simulink model "ASM_Traffic_A11"  (R2026a)
settings: Solver=ode1  StartTime=SIM.tstart.v  StopTime=SIM.tend.v  FixedStep=SIM.StepSize.v
PostLoadFcn:
  | if any(exist('dsrtsu_mdlpostloadfcn', 'file') ~= 0), dsrtsu_mdlpostloadfcn('Execute', bdroot); end
  | try, asm_mdl_postloadfcn(bdroot, 'UpdateModel', 3600); catch, disp(lasterr); end,
InitFcn:
  | , if any(exist('rtifpga_mdlclblib', 'file') ~= 0), rtifpga_mdlclblib('Init', bdroot); end,
  | , if any(exist('dsmpb_private', 'file') ~= 0), dsmpb_private('dsmpb_mdlclblib', 'Init', bdroot); end,
undefined symbols (not defined in the file): _to_, a0b2, ASM_BrakeHydraulics_DemoSystems, ASM_VehicleDynamics_DemoSystems, b98103fe8ad365046cd0, BrakeCircuit, controllerConfig, CPT, Crankshaft, DiscIntNeverNeededParam, dsmsi, FinalDriveAssembly, instance, MDL, ModeSignals, mu, Pos_BrakePedal_Maneuver, rad, RefSignals, s_to_rpm, SIM, SoftECU, Suspension, Tire, Transmission
libraries: ASM_Traffic_lib x135, simulink x98, ASM_Utils_lib x77, ASM_VehicleDynamics_lib x70, ASM_Environment_lib x22, dsmpblib x20, dsmsilib x15, MDLD_Utils_lib x10, ASM_BrakeHydraulics_lib x3, sl_discontinuities x2
(part 19 of 63)

== system ASM_Traffic_A11/Driver/Interface_In/ModelSignals/Mode_AcceleratorBrake[1Stim|2Driver]_ ==
  In1 : Inport
  DummyGain : Gain  SaturateOnIntegerOverflow=on  OutDataTypeStr=Inherit: Same as input  ParamDataTypeStr=Inherit: Same as input
  Out1 : Outport  VectorParamsAs1DForOutWhenUnconnected=off
  wires:
  In1/1 -> DummyGain/1
  DummyGain/1 -> Out1/1

== system ASM_Traffic_A11/Driver/Interface_In/ModelSignals/Mode_AdaptVelocityToRoad[1Off|2On]_ ==
  In1 : Inport
  Gain : Gain  SaturateOnIntegerOverflow=on  OutDataTypeStr=Inherit: Same as input  ParamDataTypeStr=Inherit: Same as input
  Out1 : Outport  VectorParamsAs1DForOutWhenUnconnected=off
  wires:
  In1/1 -> Gain/1
  Gain/1 -> Out1/1

== system ASM_Traffic_A11/Driver/Interface_In/ModelSignals/Mode_CurvatureCalculation[1Road|2Driver]_ ==
  In1 : Inport
  Gain : Gain  SaturateOnIntegerOverflow=on  OutDataTypeStr=Inherit: Same as input  ParamDataTypeStr=Inherit: Same as input
  Out1 : Outport  VectorParamsAs1DForOutWhenUnconnected=off
  wires:
  In1/1 -> Gain/1
  Gain/1 -> Out1/1

== system ASM_Traffic_A11/Driver/Interface_In/ModelSignals/Mode_ForceToRoad[1Off|2On]_ ==
  In1 : Inport
  Gain : Gain  SaturateOnIntegerOverflow=on  OutDataTypeStr=Inherit: Same as input  ParamDataTypeStr=Inherit: Same as input
  Out1 : Outport  VectorParamsAs1DForOutWhenUnconnected=off
  wires:
  Gain/1 -> Out1/1
  In1/1 -> Gain/1

== system ASM_Traffic_A11/Driver/Interface_In/ModelSignals/Mode_GearClutch[1Stim|2Driver|3OpenClutch|4RefGear]_ ==
  In1 : Inport
  DummyGain : Gain  SaturateOnIntegerOverflow=on  OutDataTypeStr=Inherit: Same as input  ParamDataTypeStr=Inherit: Same as input
  Out1 : Outport  VectorParamsAs1DForOutWhenUnconnected=off
  wires:
  In1/1 -> DummyGain/1
  DummyGain/1 -> Out1/1

== system ASM_Traffic_A11/Driver/Interface_In/ModelSignals/Mode_LatCtrl[1Pos|2Yaw]_ ==
  In1 : Inport
  Gain : Gain  SaturateOnIntegerOverflow=on  OutDataTypeStr=Inherit: Same as input  ParamDataTypeStr=Inherit: Same as input
  Out1 : Outport  VectorParamsAs1DForOutWhenUnconnected=off
  wires:
  Gain/1 -> Out1/1
  In1/1 -> Gain/1

== system ASM_Traffic_A11/Driver/Interface_In/ModelSignals/Mode_SelectorLever[1Stim|2Driver]_ ==
  In1 : Inport
  Gain : Gain  SaturateOnIntegerOverflow=on  OutDataTypeStr=Inherit: Same as input  ParamDataTypeStr=Inherit: Same as input
  Out1 : Outport  VectorParamsAs1DForOutWhenUnconnected=off
  wires:
  In1/1 -> Gain/1
  Gain/1 -> Out1/1

== system ASM_Traffic_A11/Driver/Interface_In/ModelSignals/Mode_Steer[1Stim|2Driver|3Fix]_ ==
  In1 : Inport
  Gain : Gain  SaturateOnIntegerOverflow=on  OutDataTypeStr=Inherit: Same as input  ParamDataTypeStr=Inherit: Same as input
  Out1 : Outport  VectorParamsAs1DForOutWhenUnconnected=off
  wires:
  In1/1 -> Gain/1
  Gain/1 -> Out1/1

== system ASM_Traffic_A11/Driver/Interface_In/ModelSignals/Mode_TrafficDriver[1Off|2On]_ ==
  In1 : Inport
  Gain : Gain  SaturateOnIntegerOverflow=on  OutDataTypeStr=Inherit: Same as input  ParamDataTypeStr=Inherit: Same as input
  Out1 : Outport  VectorParamsAs1DForOutWhenUnconnected=off
  wires:
  Gain/1 -> Out1/1
  In1/1 -> Gain/1

== system ASM_Traffic_A11/Driver/Interface_In/ModelSignals/Mode_Transmission[1Manual|2Automatic]_ ==
  In1 : Inport
  DummyGain : Gain  SaturateOnIntegerOverflow=on  OutDataTypeStr=Inherit: Same as input  ParamDataTypeStr=Inherit: Same as input
  Out1 : Outport  VectorParamsAs1DForOutWhenUnconnected=off
  wires:
  In1/1 -> DummyGain/1
  DummyGain/1 -> Out1/1

== system ASM_Traffic_A11/Driver/Interface_In/ModelSignals/Pitch_Preview_Road[deg]_ ==
  In1 : Inport
  Gain : Gain  SaturateOnIntegerOverflow=on  OutDataTypeStr=Inherit: Same as input  ParamDataTypeStr=Inherit: Same as input
  Out1 : Outport  VectorParamsAs1DForOutWhenUnconnected=off
  wires:
  Gain/1 -> Out1/1
  In1/1 -> Gain/1

== system ASM_Traffic_A11/Driver/Interface_In/ModelSignals/Pos_AccPedal_Maneuver[%]_ ==
  In1 : Inport
  DummyGain : Gain  SaturateOnIntegerOverflow=on  OutDataTypeStr=Inherit: Same as input  ParamDataTypeStr=Inherit: Same as input
  Out1 : Outport  VectorParamsAs1DForOutWhenUnconnected=off
  wires:
  In1/1 -> DummyGain/1
  DummyGain/1 -> Out1/1

== system ASM_Traffic_A11/Driver/Interface_In/ModelSignals/Pos_BrakePedal_Maneuver[%]_ ==
  In1 : Inport
  DummyGain : Gain  SaturateOnIntegerOverflow=on  OutDataTypeStr=Inherit: Same as input  ParamDataTypeStr=Inherit: Same as input
  Out1 : Outport  VectorParamsAs1DForOutWhenUnconnected=off
  wires:
  In1/1 -> DummyGain/1
  DummyGain/1 -> Out1/1

== system ASM_Traffic_A11/Driver/Interface_In/ModelSignals/Pos_ClutchPedal_Maneuver[%]_ ==
  In1 : Inport
  DummyGain : Gain  SaturateOnIntegerOverflow=on  OutDataTypeStr=Inherit: Same as input  ParamDataTypeStr=Inherit: Same as input
  Out1 : Outport  VectorParamsAs1DForOutWhenUnconnected=off
  wires:
  In1/1 -> DummyGain/1
  DummyGain/1 -> Out1/1

== system ASM_Traffic_A11/Driver/Interface_In/ModelSignals/Pos_x_CoG_Vehicle_Total[m]_ ==
  In1 : Inport
  DummyGain : Gain  SaturateOnIntegerOverflow=on  OutDataTypeStr=Inherit: Same as input  ParamDataTypeStr=Inherit: Same as input
  Out1 : Outport  VectorParamsAs1DForOutWhenUnconnected=off
  wires:
  In1/1 -> DummyGain/1
  DummyGain/1 -> Out1/1

== system ASM_Traffic_A11/Driver/Interface_In/ModelSignals/Pos_x_Preview_DriverCurv[m]_ ==
  In1 : Inport
  Gain : Gain  SaturateOnIntegerOverflow=on  OutDataTypeStr=Inherit: Same as input  ParamDataTypeStr=Inherit: Same as input
  Out1 : Outport  VectorParamsAs1DForOutWhenUnconnected=off
  wires:
  In1/1 -> Gain/1
  Gain/1 -> Out1/1

== system ASM_Traffic_A11/Driver/Interface_In/ModelSignals/Pos_x_Preview_Road[m]_ ==
  In1 : Inport
  Gain : Gain  SaturateOnIntegerOverflow=on  OutDataTypeStr=Inherit: Same as input  ParamDataTypeStr=Inherit: Same as input
  Out1 : Outport  VectorParamsAs1DForOutWhenUnconnected=off
  wires:
  Gain/1 -> Out1/1
  In1/1 -> Gain/1

== system ASM_Traffic_A11/Driver/Interface_In/ModelSignals/Pos_x_Ref_Vehicle_Road[m]_ ==
  In1 : Inport
  Gain : Gain  SaturateOnIntegerOverflow=on  OutDataTypeStr=Inherit: Same as input  ParamDataTypeStr=Inherit: Same as input
  Out1 : Outport  VectorParamsAs1DForOutWhenUnconnected=off
  wires:
  Gain/1 -> Out1/1
  In1/1 -> Gain/1

== system ASM_Traffic_A11/Driver/Interface_In/ModelSignals/Pos_x_Vehicle_CoorSys_E[m]_ ==
  In1 : Inport
  DummyGain : Gain  SaturateOnIntegerOverflow=on  OutDataTypeStr=Inherit: Same as input  ParamDataTypeStr=Inherit: Same as input
  Out1 : Outport  VectorParamsAs1DForOutWhenUnconnected=off
  wires:
  In1/1 -> DummyGain/1
  DummyGain/1 -> Out1/1

== system ASM_Traffic_A11/Driver/Interface_In/ModelSignals/Pos_y_Preview_DriverCurv[m]_ ==
  In1 : Inport
  Gain : Gain  SaturateOnIntegerOverflow=on  OutDataTypeStr=Inherit: Same as input  ParamDataTypeStr=Inherit: Same as input
  Out1 : Outport  VectorParamsAs1DForOutWhenUnconnected=off
  wires:
  Gain/1 -> Out1/1
  In1/1 -> Gain/1

== system ASM_Traffic_A11/Driver/Interface_In/ModelSignals/Pos_y_Preview_Road[m]_ ==
  In1 : Inport
  Gain : Gain  SaturateOnIntegerOverflow=on  OutDataTypeStr=Inherit: Same as input  ParamDataTypeStr=Inherit: Same as input
  Out1 : Outport  VectorParamsAs1DForOutWhenUnconnected=off
  wires:
  In1/1 -> Gain/1
  Gain/1 -> Out1/1

== system ASM_Traffic_A11/Driver/Interface_In/ModelSignals/Pos_y_Ref_Vehicle_Road[m]_ ==
  In1 : Inport
  Gain : Gain  SaturateOnIntegerOverflow=on  OutDataTypeStr=Inherit: Same as input  ParamDataTypeStr=Inherit: Same as input
  Out1 : Outport  VectorParamsAs1DForOutWhenUnconnected=off
  wires:
  In1/1 -> Gain/1
  Gain/1 -> Out1/1

== system ASM_Traffic_A11/Driver/Interface_In/ModelSignals/Pos_y_Vehicle_CoorSys_E[m]_ ==
  In1 : Inport
  DummyGain : Gain  SaturateOnIntegerOverflow=on  OutDataTypeStr=Inherit: Same as input  ParamDataTypeStr=Inherit: Same as input
  Out1 : Outport  VectorParamsAs1DForOutWhenUnconnected=off
  wires:
  DummyGain/1 -> Out1/1
  In1/1 -> DummyGain/1

== system ASM_Traffic_A11/Driver/Interface_In/ModelSignals/Pos_z_Preview_Road[m]_ ==
  In1 : Inport
  Gain : Gain  SaturateOnIntegerOverflow=on  OutDataTypeStr=Inherit: Same as input  ParamDataTypeStr=Inherit: Same as input
  Out1 : Outport  VectorParamsAs1DForOutWhenUnconnected=off
  wires:
  Gain/1 -> Out1/1
  In1/1 -> Gain/1

== system ASM_Traffic_A11/Driver/Interface_In/ModelSignals/Reset_States[0|1]_ ==
  In1 : Inport
  DummyGain : Gain  SaturateOnIntegerOverflow=on  OutDataTypeStr=Inherit: Same as input  ParamDataTypeStr=Inherit: Same as input
  Out1 : Outport  VectorParamsAs1DForOutWhenUnconnected=off
  wires:
  DummyGain/1 -> Out1/1
  In1/1 -> DummyGain/1

== system ASM_Traffic_A11/Driver/Interface_In/ModelSignals/Roll_Preview_Road[deg]_ ==
  In1 : Inport
  Gain : Gain  SaturateOnIntegerOverflow=on  OutDataTypeStr=Inherit: Same as input  ParamDataTypeStr=Inherit: Same as input
  Out1 : Outport  VectorParamsAs1DForOutWhenUnconnected=off
  wires:
  In1/1 -> Gain/1
  Gain/1 -> Out1/1

== system ASM_Traffic_A11/Driver/Interface_In/ModelSignals/Route_Direction_Init[]_ ==
  In1 : Inport
  Gain : Gain  SaturateOnIntegerOverflow=on  OutDataTypeStr=Inherit: Same as input  ParamDataTypeStr=Inherit: Same as input
  Out1 : Outport  VectorParamsAs1DForOutWhenUnconnected=off
  wires:
  Gain/1 -> Out1/1
  In1/1 -> Gain/1

== system ASM_Traffic_A11/Driver/Interface_In/ModelSignals/SelectorLever_Maneuver[-3T|-2P|-1R|0N|1D]_ ==
  In1 : Inport
  DummyGain : Gain  SaturateOnIntegerOverflow=on  OutDataTypeStr=Inherit: Same as input  ParamDataTypeStr=Inherit: Same as input
  Out1 : Outport  VectorParamsAs1DForOutWhenUnconnected=off
  wires:
  In1/1 -> DummyGain/1
  DummyGain/1 -> Out1/1

== system ASM_Traffic_A11/Driver/Interface_In/ModelSignals/Speed_Limit_Preview_Road[km|h]_ ==
  In1 : Inport
  Gain : Gain  SaturateOnIntegerOverflow=on  OutDataTypeStr=Inherit: Same as input  ParamDataTypeStr=Inherit: Same as input
  Out1 : Outport  VectorParamsAs1DForOutWhenUnconnected=off
  wires:
  In1/1 -> Gain/1
  Gain/1 -> Out1/1

== system ASM_Traffic_A11/Driver/Interface_In/ModelSignals/State_Engine[0|1|2|3|4]_ ==
  In1 : Inport
  DummyGain : Gain  SaturateOnIntegerOverflow=on  OutDataTypeStr=Inherit: Same as input  ParamDataTypeStr=Inherit: Same as input
  Out1 : Outport  VectorParamsAs1DForOutWhenUnconnected=off
  wires:
  DummyGain/1 -> Out1/1
  In1/1 -> DummyGain/1

== system ASM_Traffic_A11/Driver/Interface_In/ModelSignals/State_StartStop[1Off|2NotReady|3Ready|4EngStopped]_ ==
  In1 : Inport
  DummyGain : Gain  SaturateOnIntegerOverflow=on  OutDataTypeStr=Inherit: Same as input  ParamDataTypeStr=Inherit: Same as input
  Out1 : Outport  VectorParamsAs1DForOutWhenUnconnected=off
  wires:
  In1/1 -> DummyGain/1
  DummyGain/1 -> Out1/1

== system ASM_Traffic_A11/Driver/Interface_In/ModelSignals/Sw_LatDriver[1LatCtrl1|2LatCtrl2]_ ==
  In1 : Inport
  Gain : Gain  SaturateOnIntegerOverflow=on  OutDataTypeStr=Inherit: Same as input  ParamDataTypeStr=Inherit: Same as input
  Out1 : Outport  VectorParamsAs1DForOutWhenUnconnected=off
  wires:
  In1/1 -> Gain/1
  Gain/1 -> Out1/1

== system ASM_Traffic_A11/Driver/Interface_In/ModelSignals/Sw_ModelDeskPlottingInterface[0Disabled|1Enabled]_ ==
  In1 : Inport
  Gain : Gain
  Out1 : Outport
  wires:
  Gain/1 -> Out1/1
  In1/1 -> Gain/1

== system ASM_Traffic_A11/Driver/Interface_In/ModelSignals/Sw_ModelPortBlocks[0Disabled|1Enabled]_ ==
  In1 : Inport
  Gain : Gain
  Out1 : Outport
  wires:
  Gain/1 -> Out1/1
  In1/1 -> Gain/1

== system ASM_Traffic_A11/Driver/Interface_In/ModelSignals/Width_Deadzone_LatCtrl[m]_ ==
  In1 : Inport
  Gain : Gain  SaturateOnIntegerOverflow=on  OutDataTypeStr=Inherit: Same as input  ParamDataTypeStr=Inherit: Same as input
  Out1 : Outport  VectorParamsAs1DForOutWhenUnconnected=off
  wires:
  In1/1 -> Gain/1
  Gain/1 -> Out1/1

== system ASM_Traffic_A11/Driver/Interface_In/ModelSignals/YawRate_Vehicle[deg|s]_ ==
  In1 : Inport
  DummyGain : Gain  SaturateOnIntegerOverflow=on  OutDataTypeStr=Inherit: Same as input  ParamDataTypeStr=Inherit: Same as input
  Out1 : Outport  VectorParamsAs1DForOutWhenUnconnected=off
  wires:
  DummyGain/1 -> Out1/1
  In1/1 -> DummyGain/1

== system ASM_Traffic_A11/Driver/Interface_In/ModelSignals/a_x_Max[m|s2]_ ==
  In1 : Inport
  DummyGain : Gain  SaturateOnIntegerOverflow=on  OutDataTypeStr=Inherit: Same as input  ParamDataTypeStr=Inherit: Same as input
  Out1 : Outport  VectorParamsAs1DForOutWhenUnconnected=off
  wires:
  DummyGain/1 -> Out1/1
  In1/1 -> DummyGain/1

== system ASM_Traffic_A11/Driver/Interface_In/ModelSignals/a_x_Min[m|s2]_ ==
  In1 : Inport
  DummyGain : Gain  SaturateOnIntegerOverflow=on  OutDataTypeStr=Inherit: Same as input  ParamDataTypeStr=Inherit: Same as input
  Out1 : Outport  VectorParamsAs1DForOutWhenUnconnected=off
  wires:
  In1/1 -> DummyGain/1
  DummyGain/1 -> Out1/1

== system ASM_Traffic_A11/Driver/Interface_In/ModelSignals/a_x_Vehicle_Ref_TrafficDriver[m|s2]_ ==
  In1 : Inport
  Gain : Gain  SaturateOnIntegerOverflow=on  OutDataTypeStr=Inherit: Same as input  ParamDataTypeStr=Inherit: Same as input
  Out1 : Outport  VectorParamsAs1DForOutWhenUnconnected=off
  wires:
  Gain/1 -> Out1/1
  In1/1 -> Gain/1

== system ASM_Traffic_A11/Driver/Interface_In/ModelSignals/a_y_Max[m|s2]_ ==
  In1 : Inport
  DummyGain : Gain  SaturateOnIntegerOverflow=on  OutDataTypeStr=Inherit: Same as input  ParamDataTypeStr=Inherit: Same as input
  Out1 : Outport  VectorParamsAs1DForOutWhenUnconnected=off
  wires:
  DummyGain/1 -> Out1/1
  In1/1 -> DummyGain/1

== system ASM_Traffic_A11/Driver/Interface_In/ModelSignals/i_Steering_Mean[]_ ==
  In1 : Inport
  DummyGain : Gain  SaturateOnIntegerOverflow=on  OutDataTypeStr=Inherit: Same as input  ParamDataTypeStr=Inherit: Same as input
  Out1 : Outport  VectorParamsAs1DForOutWhenUnconnected=off
  wires:
  DummyGain/1 -> Out1/1
  In1/1 -> DummyGain/1

== system ASM_Traffic_A11/Driver/Interface_In/ModelSignals/m_Total_Vehicle[kg]_ ==
  In1 : Inport
  DummyGain : Gain  SaturateOnIntegerOverflow=on  OutDataTypeStr=Inherit: Same as input  ParamDataTypeStr=Inherit: Same as input
  Out1 : Outport  VectorParamsAs1DForOutWhenUnconnected=off
  wires:
  DummyGain/1 -> Out1/1
  In1/1 -> DummyGain/1

== system ASM_Traffic_A11/Driver/Interface_In/ModelSignals/n_Engine[rpm]_ ==
  In1 : Inport
  DummyGain : Gain  SaturateOnIntegerOverflow=on  OutDataTypeStr=Inherit: Same as input  ParamDataTypeStr=Inherit: Same as input
  Out1 : Outport  VectorParamsAs1DForOutWhenUnconnected=off
  wires:
  DummyGain/1 -> Out1/1
  In1/1 -> DummyGain/1

== system ASM_Traffic_A11/Driver/Interface_In/ModelSignals/n_Engine_Idle_Set[rpm]_ ==
  In1 : Inport
  DummyGain : Gain  SaturateOnIntegerOverflow=on  OutDataTypeStr=Inherit: Same as input  ParamDataTypeStr=Inherit: Same as input
  Out1 : Outport  VectorParamsAs1DForOutWhenUnconnected=off
  wires:
  In1/1 -> DummyGain/1
  DummyGain/1 -> Out1/1

== system ASM_Traffic_A11/Driver/Interface_In/ModelSignals/omega_Out_Trm[rad|s]_ ==
  In1 : Inport
  DummyGain : Gain  SaturateOnIntegerOverflow=on  OutDataTypeStr=Inherit: Same as input  ParamDataTypeStr=Inherit: Same as input
  Out1 : Outport  VectorParamsAs1DForOutWhenUnconnected=off
  wires:
  DummyGain/1 -> Out1/1
  In1/1 -> DummyGain/1

== system ASM_Traffic_A11/Driver/Interface_In/ModelSignals/s_Total_Vehicle_Road[m]_ ==
  In1 : Inport
  Gain : Gain  SaturateOnIntegerOverflow=on  OutDataTypeStr=Inherit: Same as input  ParamDataTypeStr=Inherit: Same as input
  Out1 : Outport  VectorParamsAs1DForOutWhenUnconnected=off
  wires:
  Gain/1 -> Out1/1
  In1/1 -> Gain/1

== system ASM_Traffic_A11/Driver/Interface_In/ModelSignals/s_Vehicle_Init[m]_ ==
  In1 : Inport
  Gain : Gain  SaturateOnIntegerOverflow=on  OutDataTypeStr=Inherit: Same as input  ParamDataTypeStr=Inherit: Same as input
  Out1 : Outport  VectorParamsAs1DForOutWhenUnconnected=off
  wires:
  Gain/1 -> Out1/1
  In1/1 -> Gain/1

== system ASM_Traffic_A11/Driver/Interface_In/ModelSignals/v_Vehicle_Preview_Ref_Maneuver[m|s]_ ==
  In1 : Inport
  DummyGain : Gain  SaturateOnIntegerOverflow=on  OutDataTypeStr=Inherit: Same as input  ParamDataTypeStr=Inherit: Same as input
  Out1 : Outport  VectorParamsAs1DForOutWhenUnconnected=off
  wires:
  In1/1 -> DummyGain/1
  DummyGain/1 -> Out1/1

== system ASM_Traffic_A11/Driver/Interface_In/ModelSignals/v_Vehicle_Ref_Maneuver[m|s]_ ==
  In1 : Inport
  DummyGain : Gain  SaturateOnIntegerOverflow=on  OutDataTypeStr=Inherit: Same as input  ParamDataTypeStr=Inherit: Same as input
  Out1 : Outport  VectorParamsAs1DForOutWhenUnconnected=off
  wires:
  DummyGain/1 -> Out1/1
  In1/1 -> DummyGain/1

== system ASM_Traffic_A11/Driver/Interface_In/ModelSignals/v_x_Vehicle[km|h]_ ==
  In1 : Inport
  DummyGain : Gain  SaturateOnIntegerOverflow=on  OutDataTypeStr=Inherit: Same as input  ParamDataTypeStr=Inherit: Same as input
  Out1 : Outport  VectorParamsAs1DForOutWhenUnconnected=off
  wires:
  DummyGain/1 -> Out1/1
  In1/1 -> DummyGain/1

== system ASM_Traffic_A11/Driver/Interface_In/ModelSignals/v_y_Vehicle[km|h]_ ==
  In1 : Inport
  DummyGain : Gain  SaturateOnIntegerOverflow=on  OutDataTypeStr=Inherit: Same as input  ParamDataTypeStr=Inherit: Same as input
  Out1 : Outport  VectorParamsAs1DForOutWhenUnconnected=off
  wires:
  In1/1 -> DummyGain/1
  DummyGain/1 -> Out1/1

== system ASM_Traffic_A11/Driver/Interface_Out/Plant_ModelSignals/Angle_SteeringWheel[deg]_ ==
  In1 : Inport
  DummyGain : Gain  SaturateOnIntegerOverflow=on  OutDataTypeStr=Inherit: Same as input  ParamDataTypeStr=Inherit: Same as input
  Out1 : Outport  VectorParamsAs1DForOutWhenUnconnected=off
  wires:
  In1/1 -> DummyGain/1
  DummyGain/1 -> Out1/1

== system ASM_Traffic_A11/Driver/Interface_Out/Plant_ModelSignals/Gear[]_ ==
  In1 : Inport
  DummyGain : Gain  SaturateOnIntegerOverflow=on  OutDataTypeStr=Inherit: Same as input  ParamDataTypeStr=Inherit: Same as input
  Out1 : Outport  VectorParamsAs1DForOutWhenUnconnected=off
  wires:
  DummyGain/1 -> Out1/1
  In1/1 -> DummyGain/1

== system ASM_Traffic_A11/Driver/Interface_Out/Plant_ModelSignals/Pos_AccPedal[%]_ ==
  In1 : Inport
  DummyGain : Gain  SaturateOnIntegerOverflow=on  OutDataTypeStr=Inherit: Same as input  ParamDataTypeStr=Inherit: Same as input
  Out1 : Outport  VectorParamsAs1DForOutWhenUnconnected=off
  wires:
  DummyGain/1 -> Out1/1
  In1/1 -> DummyGain/1

== system ASM_Traffic_A11/Driver/Interface_Out/Plant_ModelSignals/Pos_BrakePedal[%]_ ==
  In1 : Inport
  DummyGain : Gain  SaturateOnIntegerOverflow=on  OutDataTypeStr=Inherit: Same as input  ParamDataTypeStr=Inherit: Same as input
  Out1 : Outport  VectorParamsAs1DForOutWhenUnconnected=off
  wires:
  DummyGain/1 -> Out1/1
  In1/1 -> DummyGain/1

== system ASM_Traffic_A11/Driver/Interface_Out/Plant_ModelSignals/Pos_ClutchPedal[%]_ ==
  In1 : Inport
  DummyGain : Gain  SaturateOnIntegerOverflow=on  OutDataTypeStr=Inherit: Same as input  ParamDataTypeStr=Inherit: Same as input
  Out1 : Outport  VectorParamsAs1DForOutWhenUnconnected=off
  wires:
  DummyGain/1 -> Out1/1
  In1/1 -> DummyGain/1

== system ASM_Traffic_A11/Driver/Interface_Out/Plant_ModelSignals/SelectorLever[-3T|-2P|-1R|0N|1D]_ ==
  In1 : Inport
  DummyGain : Gain  SaturateOnIntegerOverflow=on  OutDataTypeStr=Inherit: Same as input  ParamDataTypeStr=Inherit: Same as input
  Out1 : Outport  VectorParamsAs1DForOutWhenUnconnected=off
  wires:
  DummyGain/1 -> Out1/1
  In1/1 -> DummyGain/1

== system ASM_Traffic_A11/Driver/Interface_Out/Plant_ModelSignals/s_Preview[m]_ ==
  In1 : Inport
  DummyGain : Gain  SaturateOnIntegerOverflow=on  OutDataTypeStr=Inherit: Same as input  ParamDataTypeStr=Inherit: Same as input
  Out1 : Outport  VectorParamsAs1DForOutWhenUnconnected=off
  wires:
  In1/1 -> DummyGain/1
  DummyGain/1 -> Out1/1

== system ASM_Traffic_A11/Driver/Interface_Out/Plant_ModelSignals/t_Preview_vRef_Driver[s]_ ==
  In1 : Inport
  DummyGain : Gain  SaturateOnIntegerOverflow=on  OutDataTypeStr=Inherit: Same as input  ParamDataTypeStr=Inherit: Same as input
  Out1 : Outport  VectorParamsAs1DForOutWhenUnconnected=off
  wires:
  In1/1 -> DummyGain/1
  DummyGain/1 -> Out1/1

== system ASM_Traffic_A11/Driver/Plant/Driver/ASMSignalCollector ==
  Bus Creator : BusCreator  Inputs=2
  Bus Creator1 : BusCreator  Inputs=4
  Bus Creator2 : BusCreator  Inputs=3
  Bus Creator3 : BusCreator  Inputs=2
  ASMSignalBus : Outport  VectorParamsAs1DForOutWhenUnconnected=off
  wires:
  Bus Creator3/1 -> Bus Creator1/3  "ReferenceVelocity"
  [ASMBUS_Driver_Curvature] -> Bus Creator3/2
  [ASMBUS_Driver_SpeedProfiler] -> Bus Creator3/1
  [ASMBUS_Driver_LatCtrl1] -> Bus Creator2/1
  [ASMBUS_Driver_LatCtrl2] -> Bus Creator2/2
  Bus Creator2/1 -> Bus Creator1/2  "LateralController"
  [ASMBUS_Driver_LatCtrl_PosError] -> Bus Creator2/3
  Bus Creator/1 -> Bus Creator1/1  "LongitudinalController"
  [ASMBUS_Driver_GearShifter] -> Bus Creator/2
  [ASMBUS_Driver_LongCtrl] -> Bus Creator/1
  Bus Creator1/1 -> ASMSignalBus/1  "Plant"
  [ASMBUS_Driver_OutputSignals] -> Bus Creator1/4

== system ASM_Traffic_A11/Driver/Plant/Driver/LateralController ==
  Interface_In : Inport
  Bus Selector1 : BusSelector  OutputSignals=ExternalModel.v_x_Vehicle[km|h],ExternalModel.v_y_Vehicle[km|h],ExternalModel.Angle_Yaw_Vehicle_CoorSys_E[deg],ExternalModel.YawRate_Vehicle[deg|s],ExternalModel.Pos_x_Vehicle_CoorSys_E[m],ExternalModel.Pos_y_Vehicle_CoorSys_E[m],ExternalModel.i_Steering_Mean[],ExternalModel.CorneringStiffness_Tire_Front[N|rad],ExternalModel.CorneringStiffness_Tire_Rear[N|rad],ExternalModel.Pos_x_Preview_Road[m],ExternalModel.Pos_y_Preview_Road[m]
  Bus Selector3 : BusSelector  OutputSignals=ExternalModel.m_Total_Vehicle[kg],ExternalModel.Pos_x_CoG_Vehicle_Total[m],ExternalModel.Inertia_z_Vehicle_Total[kgm2],ExternalModel.Width_Deadzone_LatCtrl[m],ExternalModel.Reset_States[0|1],ExternalModel.Mode_Steer[1Stim|2Driver|3Fix],ExternalModel.Angle_SteeringWheel_Maneuver[deg]
  Bus Selector4 : BusSelector  OutputSignals=ExternalModel.i_Steering_Mean[],ExternalModel.v_x_Vehicle[km|h],ExternalModel.Angle_Yaw_Vehicle_CoorSys_E[deg],ExternalModel.Pos_x_Vehicle_CoorSys_E[m],ExternalModel.Pos_y_Vehicle_CoorSys_E[m],ExternalModel.Angle_Yaw_Veh_Road[deg],ExternalModel.Pos_x_Ref_Vehicle_Road[m],ExternalModel.Pos_x_Preview_Road[m],ExternalModel.Pos_y_Ref_Vehicle_Road[m],ExternalModel.Pos_y_Preview_Road[m]
  Bus Selector5 : BusSelector  OutputSignals=ExternalModel.Width_Deadzone_LatCtrl[m],ExternalModel.Reset_States[0|1],ExternalModel.Mode_Steer[1Stim|2Driver|3Fix],ExternalModel.Angle_SteeringWheel_Maneuver[deg],ExternalModel.YawRate_Vehicle[deg|s],ExternalModel.Mode_LatCtrl[1Pos|2Yaw],ExternalModel.Curv_Veh_Road[1|m]
  Bus Selector6 : BusSelector  OutputSignals=ExternalModel.Sw_LatDriver[1LatCtrl1|2LatCtrl2]
  Bus Selector7 : BusSelector  OutputSignals=ExternalModel.Angle_Yaw_Vehicle_CoorSys_E[deg],ExternalModel.Pos_x_Vehicle_CoorSys_E[m],ExternalModel.Pos_y_Vehicle_CoorSys_E[m],ExternalModel.Pos_x_Ref_Vehicle_Road[m],ExternalModel.Pos_y_Ref_Vehicle_Road[m]
  LATERAL_CONTROL1 : ASM_Environment_lib/Environment/Driver/LATERAL_CONTROL1  Tag=ASM_SUBCOMPONENT  Const_t_Preview_LatCtrl=MDL.Environment.Driver.LateralController.LateralControl1.Const_t_Preview_LatCtrl  Const_t_PT1_LatCtrl=MDL.Environment.Driver.LateralController.LateralControl1.Const_t_PT1_LatCtrl  Const_WheelBase=MDL.Environment.Driver.LateralController.LateralControl1.Const_WheelBase  StepSize=SIM.StepSize  ASMProperties=struct('Name','LATERAL_CONTROL1','Version','15.0','Library','ASM_Environment_lib')  ASMInstanceName=lateral_control1  ASMInstanceID=1
  LATERAL_CONTROL2 : ASM_Environment_lib/Environment/Driver/LATERAL_CONTROL2  Tag=ASM_SUBCOMPONENT  Const_LatCtrl_kLat=MDL.Environment.Driver.LateralController.LateralControl2.Const_LatCtrl_kLat  Const_LatCtrl_kLat_i=MDL.Environment.Driver.LateralController.LateralControl2.Const_LatCtrl_kLat_i  Const_LatCtrl_kLat_Preview=MDL.Environment.Driver.LateralController.LateralControl2.Const_LatCtrl_kLat_Preview  Const_LatCtrl_kYaw=MDL.Environment.Driver.LateralController.LateralControl2.Const_LatCtrl_kYaw  Const_t_Preview_LatCtrl=MDL.Environment.Driver.LateralController.LateralControl2.Const_t_Preview_LatCtrl  Const_t_PT1_LatCtrl=MDL.Environment.Driver.LateralController.LateralControl2.Const_t_PT1_LatCtrl  Const_Kp_YawRate_Ctrl=MDL.Environment.Driver.LateralController.LateralControl2.Const_Kp_YawRate_Ctrl  Const_Ki_YawRate_Ctrl=MDL.Environment.Driver.LateralController.LateralControl2.Const_Ki_YawRate_Ctrl  StepSize=SIM.StepSize  ASMProperties=struct('Name','LATERAL_CONTROL2','Version','9.0','Library','ASM_Environment_lib')  ASMInstanceName=lateral_control2  ASMInstanceID=1
  LatCtrl1_Enable : Subsystem
  LatCtrl2_Enable : Subsystem
  Memory : Memory
  Multiport Switch : MultiPortSwitch  Inputs=2  InputSameDT=off
  Multiport Switch1 : MultiPortSwitch  Inputs=2  InputSameDT=off
  POSITION_ERRORS : ASM_Environment_lib/Environment/Driver/POSITION_ERRORS  Tag=ASM_SUBCOMPONENT  ASMProperties=struct('Name','POSITION_ERRORS','Version','2.0','Library','ASM_Environment_lib')  ASMInstanceName=position_errors  ASMInstanceID=1
  Terminator : Terminator
  UnitConversion1 : ASM_Utils_lib/UnitConversion/UnitConversion  Selection=km/h_to_m/s
  UnitConversion2 : ASM_Utils_lib/UnitConversion/UnitConversion  Selection=km/h_to_m/s
  UnitConversion3 : ASM_Utils_lib/UnitConversion/UnitConversion  Selection=deg_to_rad
  UnitConversion4 : ASM_Utils_lib/UnitConversion/UnitConversion  Selection=km/h_to_m/s
  UnitConversion5 : ASM_Utils_lib/UnitConversion/UnitConversion  Selection=deg_to_rad
  s_Preview_LatCtrl[m] : Outport  VectorParamsAs1DForOutWhenUnconnected=off
  Angle_SteeringWheel[deg] : Outport  Port=2  VectorParamsAs1DForOutWhenUnconnected=off
  tag scope: ASMBUS_Driver_LatCtrl1=scoped, ASMBUS_Driver_LatCtrl2=scoped, ASMBUS_Driver_LatCtrl_PosError=scoped
  wires:
  Bus Selector4/1 -> LATERAL_CONTROL2/2  "<i_Steering_Mean[]>"
  Bus Selector4/2 -> UnitConversion4/1  "<v_x_Vehicle[km|h]>"
  Bus Selector4/3 -> LATERAL_CONTROL2/4  "<Angle_Yaw_Vehicle_CoorSys_E[deg]>"
  Bus Selector4/4 -> LATERAL_CONTROL2/5  "<Pos_x_Vehicle_CoorSys_E[m]>"
  Bus Selector4/5 -> LATERAL_CONTROL2/6  "<Pos_y_Vehicle_CoorSys_E[m]>"
  Bus Selector7/5 -> POSITION_ERRORS/5  "<Pos_y_Ref_Vehicle_Road[m]>"
  Bus Selector7/4 -> POSITION_ERRORS/4  "<Pos_x_Ref_Vehicle_Road[m]>"
  Bus Selector7/1 -> POSITION_ERRORS/1  "<Angle_Yaw_Vehicle_CoorSys_E[deg]>"
  Bus Selector7/3 -> POSITION_ERRORS/3  "<Pos_y_Vehicle_CoorSys_E[m]>"
  Bus Selector7/2 -> POSITION_ERRORS/2  "<Pos_x_Vehicle_CoorSys_E[m]>"
  Bus Selector5/7 -> LATERAL_CONTROL2/19  "<Curv_Veh_Road[1|m]>"
  UnitConversion5/1 -> LATERAL_CONTROL2/17
  Bus Selector5/5 -> UnitConversion5/1  "<YawRate_Vehicle[deg|s]>"
  Bus Selector5/6 -> LATERAL_CONTROL2/18  "<Mode_LatCtrl[1Pos|2Yaw]>"
  Bus Selector5/4 -> LATERAL_CONTROL2/16  "<Angle_SteeringWheel_Maneuver[deg]>"
  Bus Selector5/3 -> LATERAL_CONTROL2/15  "<Mode_Steer[1Stim|2Driver|3Fix]>"
  Bus Selector5/1 -> LATERAL_CONTROL2/13  "<Width_Deadzone_LatCtrl[m]>"
  Bus Selector5/2 -> LATERAL_CONTROL2/14  "<Reset_States[0|1]>"
  Bus Selector3/3 -> LATERAL_CONTROL1/16  "<Inertia_z_Vehicle_Total[kgm2]>"
  Bus Selector3/2 -> LATERAL_CONTROL1/15  "<Pos_x_CoG_Vehicle_Total[m]>"
  Bus Selector3/1 -> LATERAL_CONTROL1/14  "<m_Total_Vehicle[kg]>"
  Bus Selector1/11 -> LATERAL_CONTROL1/12  "<Pos_y_Preview_Road[m]>"
  Bus Selector1/10 -> LATERAL_CONTROL1/11  "<Pos_x_Preview_Road[m]>"
  UnitConversion4/1 -> LATERAL_CONTROL2/3
  LatCtrl1_Enable/1(Out1) -> LATERAL_CONTROL1/1
  Bus Selector1/9 -> LATERAL_CONTROL1/10  "<CorneringStiffness_Tire_Rear[N|rad]>"
  Bus Selector1/8 -> LATERAL_CONTROL1/9  "<CorneringStiffness_Tire_Front[N|rad]>"
  Bus Selector1/7 -> LATERAL_CONTROL1/8  "<i_Steering_Mean[]>"
  Bus Selector1/6 -> LATERAL_CONTROL1/7  "<Pos_y_Vehicle_CoorSys_E[m]>"
  Bus Selector1/5 -> LATERAL_CONTROL1/6  "<Pos_x_Vehicle_CoorSys_E[m]>"
  Bus Selector1/4 -> UnitConversion3/1  "<YawRate_Vehicle[deg|s]>"
  Bus Selector1/3 -> LATERAL_CONTROL1/4  "<Angle_Yaw_Vehicle_CoorSys_E[deg]>"
  Bus Selector1/2 -> UnitConversion2/1  "<v_y_Vehicle[km|h]>"
  Bus Selector1/1 -> UnitConversion1/1  "<v_x_Vehicle[km|h]>"
  Bus Selector6/1 -> Multiport Switch1/1, Multiport Switch/1  "<Sw_LatDriver[1LatCtrl1|2LatCtrl2]>"
  Interface_In/1 -> Bus Selector6/1, LatCtrl1_Enable/1(Interface_In), Bus Selector1/1, Bus Selector3/1, LatCtrl2_Enable/1(Interface_In), Bus Selector7/1, Bus Selector5/1, Bus Selector4/1
  LATERAL_CONTROL1/1 -> [ASMBUS_Driver_LatCtrl1]
  Bus Selector4/8 -> LATERAL_CONTROL2/9  "<Pos_x_Preview_Road[m]>"
  Bus Selector4/10 -> LATERAL_CONTROL2/11  "<Pos_y_Preview_Road[m]>"
  Multiport Switch/1 -> s_Preview_LatCtrl[m]/1
  LATERAL_CONTROL2/2 -> Multiport Switch/3
  LATERAL_CONTROL1/2 -> Multiport Switch/2
  LATERAL_CONTROL1/3 -> Multiport Switch1/2
  Bus Selector4/7 -> LATERAL_CONTROL2/8  "<Pos_x_Ref_Vehicle_Road[m]>"
  Bus Selector4/9 -> LATERAL_CONTROL2/10  "<Pos_y_Ref_Vehicle_Road[m]>"
  UnitConversion2/1 -> LATERAL_CONTROL1/3
  LATERAL_CONTROL2/3 -> Multiport Switch1/3
  LATERAL_CONTROL2/1 -> [ASMBUS_Driver_LatCtrl2]
  POSITION_ERRORS/2 -> Terminator/1
  POSITION_ERRORS/1 -> [ASMBUS_Driver_LatCtrl_PosError]
  UnitConversion1/1 -> LATERAL_CONTROL1/2
  UnitConversion3/1 -> LATERAL_CONTROL1/5
  Multiport Switch1/1 -> Angle_SteeringWheel[deg]/1, Memory/1
  Memory/1 -> LATERAL_CONTROL1/13, LATERAL_CONTROL2/12
  Bus Selector3/4 -> LATERAL_CONTROL1/17  "<Width_Deadzone_LatCtrl[m]>"
  Bus Selector3/5 -> LATERAL_CONTROL1/18  "<Reset_States[0|1]>"
  Bus Selector3/6 -> LATERAL_CONTROL1/19  "<Mode_Steer[1Stim|2Driver|3Fix]>"
  Bus Selector3/7 -> LATERAL_CONTROL1/20  "<Angle_SteeringWheel_Maneuver[deg]>"
  Bus Selector4/6 -> LATERAL_CONTROL2/7  "<Angle_Yaw_Veh_Road[deg]>"
  LatCtrl2_Enable/1(Out1) -> LATERAL_CONTROL2/1

== system ASM_Traffic_A11/Driver/Plant/Driver/LongitudinalController ==
  Interface_In : Inport
  v_Vehicle_Ref[m|s] : Inport  Port=2
  v_Vehicle_Ref_Preview[m|s] : Inport  Port=3
  Bus Selector1 : BusSelector  OutputSignals=ExternalModel.v_x_Vehicle[km|h]
  Bus Selector2 : BusSelector  OutputSignals=ExternalModel.Gear_Max[0Off|1_n],ExternalModel.Pos_AccPedal_Maneuver[%],ExternalModel.Pos_BrakePedal_Maneuver[%],ExternalModel.Mode_AcceleratorBrake[1Stim|2Driver],ExternalModel.Gear_Maneuver[],ExternalModel.Pos_ClutchPedal_Maneuver[%],ExternalModel.Mode_GearClutch[1Stim|2Driver|3OpenClutch|4RefGear],ExternalModel.SelectorLever_Maneuver[-3T|-2P|-1R|0N|1D],ExternalModel.Mode_SelectorLever[1Stim|2Driver],ExternalModel.Reset_States[0|1],ExternalModel.State_StartStop[1Off|2NotReady|3Ready|4EngStopped],ExternalModel.Enable_v_Init[0|1]
  Bus Selector3 : BusSelector  OutputSignals=ExternalModel.Mode_AcceleratorBrake[1Stim|2Driver],ExternalModel.Pos_AccPedal_Maneuver[%],ExternalModel.Pos_BrakePedal_Maneuver[%],ExternalModel.Reset_States[0|1]
  Bus Selector4 : BusSelector  OutputSignals=ExternalModel.F_Driving_Res[N],ExternalModel.v_x_Vehicle[km|h]
  Bus Selector5 : BusSelector  OutputSignals=ExternalModel.State_StartStop[1Off|2NotReady|3Ready|4EngStopped],ExternalModel.Enable_v_Init[0|1]
  Bus Selector6 : BusSelector  OutputSignals=ExternalModel.n_Engine[rpm],ExternalModel.m_Total_Vehicle[kg],ExternalModel.omega_Out_Trm[rad|s],ExternalModel.State_Engine[0|1|2|3|4],ExternalModel.n_Engine_Idle_Set[rpm]
  Bus Selector7 : BusSelector  OutputSignals=ExternalModel.Mode_Transmission[1Manual|2Automatic]
  Default_GearClutch_Mode : Subsystem
      mask Display: disp('Default GearClutch_Mode')
  GEAR_SHIFTER : ASM_Environment_lib/Environment/Driver/GEAR_SHIFTER  Tag=ASM_SUBCOMPONENT  Map_Gear_StartUp=MDL.Environment.Driver.LongitudinalController.GearShifter.Map_Gear_StartUp  Const_n_Engine_StartUp_Set=MDL.Environment.Driver.LongitudinalController.GearShifter.Const_n_Engine_StartUp_Set  Const_P_Gain_StartUp=MDL.Environment.Driver.LongitudinalController.GearShifter.Const_P_Gain_StartUp  Const_I_Gain_StartUp=MDL.Environment.Driver.LongitudinalController.GearShifter.Const_I_Gain_StartUp  Const_D_Gain_StartUp=MDL.Environment.Driver.LongitudinalController.GearShifter.Const_D_Gain_StartUp  Const_a_x_Vehicle_UpLim=MDL.Environment.Driver.LongitudinalController.GearShifter.Const_a_x_Vehicle_UpLim  Const_a_Tractive_Res_UpLim=MDL.Environment.Driver.LongitudinalController.GearShifter.Const_a_Tractive_Res_UpLim  Const_v_x_Vehicle_LowLim=MDL.Environment.Driver.LongitudinalController.GearShifter.Const_v_x_Vehicle_LowLim  Const_a_x_Vehicle_LowLim=MDL.Environment.Driver.LongitudinalController.GearShifter.Const_a_x_Vehicle_LowLim  Const_t_Gear_Neutral=MDL.Environment.Driver.LongitudinalController.GearShifter.Const_t_Gear_Neutral  Const_t_Hold_ClutchPedal=MDL.Environment.Driver.LongitudinalController.GearShifter.Const_t_Hold_ClutchPedal  Map_Pos_AccPedal=MDL.Environment.Driver.LongitudinalController.GearShifter.Map_Pos_AccPedal  Const_P_Gain_ClutchPedal=MDL.Environment.Driver.LongitudinalController.GearShifter.Const_P_Gain_ClutchPedal  Const_I_Gain_ClutchPedal=MDL.Environment.Driver.LongitudinalController.GearShifter.Const_I_Gain_ClutchPedal  Map_Pos_ClutchPedal_Disengagement_StartUp=MDL.Environment.Driver.LongitudinalController.GearShifter.Map_Pos_ClutchPedal_Disengagement_StartUp  Map_Pos_ClutchPedal_Disengagement=MDL.Environment.Driver.LongitudinalController.GearShifter.Map_Pos_ClutchPedal_Disengagement  Map_Pos_ClutchPedal_Engagement_StartUp=MDL.Environment.Driver.LongitudinalController.GearShifter.Map_Pos_ClutchPedal_Engagement_StartUp  Map_Pos_ClutchPedal_Engagement=MDL.Environment.Driver.LongitudinalController.GearShifter.Map_Pos_ClutchPedal_Engagement  Map_n_Engine_Upshift_Lim=MDL.Environment.Driver.LongitudinalController.GearShifter.Map_n_Engine_Upshift_Lim  Map_n_Engine_Downshift_Lim=MDL.Environment.Driver.LongitudinalController.GearShifter.Map_n_Engine_Downshift_Lim  Map_omega_Out_Trm_Shift_Bias=MDL.Environment.Driver.LongitudinalController.GearShifter.Map_omega_Out_Trm_Shift_Bias  Map_i_Ratio=MDL.Environment.Driver.LongitudinalController.GearShifter.Map_i_Ratio  Sw_Upshift_Gear_Skipping=MDL.Environment.Driver.LongitudinalController.GearShifter.Sw_Upshift_Gear_Skipping  Sw_ClutchPedal_EngineOff=MDL.Environment.Driver.LongitudinalController.GearShifter.Sw_ClutchPedal_EngineOff  StepSize=SIM.StepSize  ASMProperties=struct('Name','GEAR_SHIFTER','Version','18.0','Library','ASM_Environment_lib')  ASMInstanceName=gear_shifter  ASMInstanceID=1
  Gain : Gain  Gain=-1
  Gear_Min_Maneuver[0Off|-n_-1] : Constant  Value=0
  LONGITUDINAL_CONTROL : ASM_Environment_lib/Environment/Driver/LONGITUDINAL_CONTROL  Tag=ASM_SUBCOMPONENT  Map_P_vCtrl=MDL.Environment.Driver.LongitudinalController.LongControl.Map_P_vCtrl  Map_I_vCtrl=MDL.Environment.Driver.LongitudinalController.LongControl.Map_I_vCtrl  Const_P_FeedForward_aCtrl=MDL.Environment.Driver.LongitudinalController.LongControl.Const_P_FeedForward_aCtrl  Const_Pos_BrakePedal_Standstill=MDL.Environment.Driver.LongitudinalController.LongControl.Const_Pos_BrakePedal_Standstill  Const_t_Min_Pedals=MDL.Environment.Driver.LongitudinalController.LongControl.Const_t_Min_Pedals  Const_Max_AccPedal=MDL.Environment.Driver.LongitudinalController.LongControl.Const_Max_AccPedal  Const_Rate_Rise_Max_AccPedal=MDL.Environment.Driver.LongitudinalController.LongControl.Const_Rate_Rise_Max_AccPedal  Const_Rate_Drop_Max_AccPedal=MDL.Environment.Driver.LongitudinalController.LongControl.Const_Rate_Drop_Max_AccPedal  Const_Max_BrakePedal=MDL.Environment.Driver.LongitudinalController.LongControl.Const_Max_BrakePedal  Const_Rate_Rise_Max_BrakePedal=MDL.Environment.Driver.LongitudinalController.LongControl.Const_Rate_Rise_Max_BrakePedal  Const_Rate_Drop_Max_BrakePedal=MDL.Environment.Driver.LongitudinalController.LongControl.Const_Rate_Drop_Max_BrakePedal  Const_t_Preview=MDL.Environment.Driver.LongitudinalController.LongControl.Const_t_Preview  StepSize=SIM.StepSize  ASMProperties=struct('Name','LONGITUDINAL_CONTROL','Version','13.0','Library','ASM_Environment_lib')  ASMInstanceName=longitudinal_control  ASMInstanceID=1
  Running_Engine : Constant  Value=3
  UnitConversion1 : ASM_Utils_lib/UnitConversion/UnitConversion  Selection=km/h_to_m/s
  UnitConversion2 : ASM_Utils_lib/UnitConversion/UnitConversion  Selection=km/h_to_m/s
  t_Preview_vRef[s] : Outport  VectorParamsAs1DForOutWhenUnconnected=off
  Pos_AccPedal[%] : Outport  Port=2  VectorParamsAs1DForOutWhenUnconnected=off
  Pos_BrakePedal[%] : Outport  Port=3  VectorParamsAs1DForOutWhenUnconnected=off
  Pos_ClutchPedal[%] : Outport  Port=4  VectorParamsAs1DForOutWhenUnconnected=off
  Gear[] : Outport  Port=5  VectorParamsAs1DForOutWhenUnconnected=off
  SelectorLever[-3T|-2P|-1R|0N|1D] : Outport  Port=6  VectorParamsAs1DForOutWhenUnconnected=off
  tag scope: ASMBUS_Driver_GearShifter=scoped, ASMBUS_Driver_LongCtrl=scoped
  wires:
  Gain/1 -> GEAR_SHIFTER/4
  Bus Selector4/2 -> UnitConversion1/1  "<v_x_Vehicle[km|h]>"
  UnitConversion1/1 -> GEAR_SHIFTER/5
  Bus Selector4/1 -> Gain/1  "<F_Driving_Res[N]>"
  Bus Selector2/11 -> GEAR_SHIFTER/23  "<State_StartStop[1Off|2NotReady|3Ready|4EngStopped]>"
  Bus Selector2/10 -> GEAR_SHIFTER/22  "<Reset_States[0|1]>"
  Bus Selector3/4 -> LONGITUDINAL_CONTROL/7  "<Reset_States[0|1]>"
  Running_Engine/1 -> LONGITUDINAL_CONTROL/8
  UnitConversion2/1 -> LONGITUDINAL_CONTROL/1
  Bus Selector6/4 -> GEAR_SHIFTER/10  "<State_Engine[0|1|2|3|4]>"
  Interface_In/1 -> Bus Selector1/1, Bus Selector7/1, Bus Selector4/1, Bus Selector6/1, Bus Selector2/1, Bus Selector5/1, Bus Selector3/1
  Bus Selector7/1 -> GEAR_SHIFTER/1, Default_GearClutch_Mode/1(Mode_Transmission[1|2])  "<Mode_Transmission[1Manual|2Automatic]>"
  Bus Selector2/9 -> GEAR_SHIFTER/21  "<Mode_SelectorLever[1Stim|2Driver]>"
  Bus Selector2/8 -> GEAR_SHIFTER/20  "<SelectorLever_Maneuver[-3T|-2P|-1R|0N|1D]>"
  Bus Selector2/7 -> Default_GearClutch_Mode/2(GearClutch_Mode[1Stim|2Driver|3OpenClutch|4RefGear])  "<Mode_GearClutch[1Stim|2Driver|3OpenClutch|4RefGear]>"
  Bus Selector2/6 -> GEAR_SHIFTER/18  "<Pos_ClutchPedal_Maneuver[%]>"
  Bus Selector2/5 -> GEAR_SHIFTER/17  "<Gear_Maneuver[]>"
  Bus Selector2/4 -> GEAR_SHIFTER/16  "<Mode_AcceleratorBrake[1Stim|2Driver]>"
  Bus Selector6/5 -> GEAR_SHIFTER/11  "<n_Engine_Idle_Set[rpm]>"
  Bus Selector6/3 -> GEAR_SHIFTER/9  "<omega_Out_Trm[rad|s]>"
  Bus Selector6/2 -> GEAR_SHIFTER/8  "<m_Total_Vehicle[kg]>"
  Bus Selector6/1 -> GEAR_SHIFTER/7  "<n_Engine[rpm]>"
  Bus Selector2/3 -> GEAR_SHIFTER/15  "<Pos_BrakePedal_Maneuver[%]>"
  Bus Selector2/2 -> GEAR_SHIFTER/14  "<Pos_AccPedal_Maneuver[%]>"
  GEAR_SHIFTER/6 -> SelectorLever[-3T|-2P|-1R|0N|1D]/1
  GEAR_SHIFTER/5 -> Gear[]/1
  GEAR_SHIFTER/4 -> Pos_ClutchPedal[%]/1
  GEAR_SHIFTER/3 -> Pos_BrakePedal[%]/1
  GEAR_SHIFTER/2 -> Pos_AccPedal[%]/1
  GEAR_SHIFTER/1 -> [ASMBUS_Driver_GearShifter]
  Bus Selector2/1 -> GEAR_SHIFTER/13  "<Gear_Max[0Off|1_n]>"
  v_Vehicle_Ref[m|s]/1 -> GEAR_SHIFTER/6, LONGITUDINAL_CONTROL/2
  Bus Selector1/1 -> UnitConversion2/1  "<v_x_Vehicle[km|h]>"
  Gear_Min_Maneuver[0Off|-n_-1]/1 -> GEAR_SHIFTER/12
  Bus Selector3/3 -> LONGITUDINAL_CONTROL/6  "<Pos_BrakePedal_Maneuver[%]>"
  Bus Selector3/2 -> LONGITUDINAL_CONTROL/5  "<Pos_AccPedal_Maneuver[%]>"
  Bus Selector3/1 -> LONGITUDINAL_CONTROL/4  "<Mode_AcceleratorBrake[1Stim|2Driver]>"
  LONGITUDINAL_CONTROL/3 -> GEAR_SHIFTER/2
  LONGITUDINAL_CONTROL/4 -> GEAR_SHIFTER/3
  LONGITUDINAL_CONTROL/2 -> t_Preview_vRef[s]/1
  LONGITUDINAL_CONTROL/1 -> [ASMBUS_Driver_LongCtrl]
  v_Vehicle_Ref_Preview[m|s]/1 -> GEAR_SHIFTER/24, LONGITUDINAL_CONTROL/3
  Default_GearClutch_Mode/1(GearClutch_Mode[1Stim|2Driver|3OpenClutch|4RefGear]_) -> GEAR_SHIFTER/19
  Bus Selector5/1 -> LONGITUDINAL_CONTROL/9  "<State_StartStop[1Off|2NotReady|3Ready|4EngStopped]>"
  Bus Selector5/2 -> LONGITUDINAL_CONTROL/10  "<Enable_v_Init[0|1]>"
  Bus Selector2/12 -> GEAR_SHIFTER/25  "<Enable_v_Init[0|1]>"

== system ASM_Traffic_A11/Driver/Plant/Driver/OutputSignals ==
  Pos_AccPedal[%] : Inport
  Pos_BrakePedal[%] : Inport  Port=2
  Pos_ClutchPedal[%] : Inport  Port=3
  Gear[] : Inport  Port=4
  SelectorLever[-3T|-2P|-1R|0N|1D] : Inport  Port=5
  s_Preview_vRef[m] : Inport  Port=6
  s_Preview_LatCtrl[m] : Inport  Port=7
  Angle_SteeringWheel[deg] : Inport  Port=8
  Bus Creator1 : BusCreator  Inputs=9
  Mux : Mux  Inputs=2
  tag scope: ASMBUS_Driver_OutputSignals=scoped
  wires:
  Mux/1 -> Bus Creator1/8  "s_Preview[m]"
  s_Preview_LatCtrl[m]/1 -> Mux/2, Bus Creator1/7  "s_Preview_LatCtrl[m]"
  s_Preview_vRef[m]/1 -> Mux/1, Bus Creator1/6  "s_Preview_vRef[m]"
  Angle_SteeringWheel[deg]/1 -> Bus Creator1/9  "Angle_SteeringWheel[deg]"
  SelectorLever[-3T|-2P|-1R|0N|1D]/1 -> Bus Creator1/5  "SelectorLever[-3T|-2P|-1R|0N|1D]"
  Gear[]/1 -> Bus Creator1/4  "Gear[]"
  Pos_ClutchPedal[%]/1 -> Bus Creator1/3  "Pos_ClutchPedal[%]"
  Pos_BrakePedal[%]/1 -> Bus Creator1/2  "Pos_BrakePedal[%]"
  Pos_AccPedal[%]/1 -> Bus Creator1/1  "Pos_AccPedal[%]"
  Bus Creator1/1 -> [ASMBUS_Driver_OutputSignals]  "OutputSignals"

== system ASM_Traffic_A11/Driver/Plant/Driver/ReferenceVelocity ==
  Interface_In : Inport
  t_Preview_vRef[s] : Inport  Port=2
  AdaptationForNegativeSpeed : Subsystem
      mask Display: disp('Adaptation for -ve Speed')
  Bus Selector2 : BusSelector  OutputSignals=ExternalModel.Mode_CurvatureCalculation[1Road|2Driver],ExternalModel.Pos_x_Preview_DriverCurv[m],ExternalModel.Pos_y_Preview_DriverCurv[m],ExternalModel.Curv_Veh_Road[1|m],ExternalModel.Curv_Preview_Road[1|m]
  Bus Selector3 : BusSelector  OutputSignals=ExternalModel.a_x_Max[m|s2],ExternalModel.a_x_Min[m|s2],ExternalModel.a_y_Max[m|s2]
  Bus Selector4 : BusSelector  OutputSignals=ExternalModel.v_x_Vehicle[km|h],ExternalModel.s_Total_Vehicle_Road[m],ExternalModel.Speed_Limit_Preview_Road[km|h],ExternalModel.Pitch_Preview_Road[deg],ExternalModel.Pos_z_Preview_Road[m],ExternalModel.Dist_Border_Left[m],ExternalModel.Dist_Border_Right[m],ExternalModel.Mode_AdaptVelocityToRoad[1Off|2On],ExternalModel.Mode_AcceleratorBrake[1Stim|2Driver],ExternalModel.v_Vehicle_Ref_Maneuver[m|s],ExternalModel.v_Vehicle_Preview_Ref_Maneuver[m|s],ExternalModel.s_Vehicle_Init[m],ExternalModel.Route_Direction_Init[],ExternalModel.Reset_States[0|1],ExternalModel.Mode_TrafficDriver[1Off|2On],ExternalModel.a_x_Vehicle_Ref_TrafficDriver[m|s2],ExternalModel.Enable_v_Init[0|1],ExternalModel.Lane_ID_Vehicle[]
  DRIVER_CURVATURE : ASM_Environment_lib/Environment/Driver/DRIVER_CURVATURE  Tag=ASM_SUBCOMPONENT  ASMProperties=struct('Name','DRIVER_CURVATURE','Version','1.0','Library','ASM_Environment_lib')  ASMInstanceName=driver_curvature  ASMInstanceID=1
  Dist_OutsideRoad_Margin[m] : Constant  Value=2
  Driver_Parameters : Subsystem
  Extend_Previews : Subsystem
  Reduce_Dimension : Subsystem
  Reduce_Dimension1 : Subsystem
  Reduce_Dimension2 : Subsystem
  Reduce_Dimension3 : Subsystem
  Reduce_Dimension4 : Subsystem
  SPEED_PROFILER : ASM_Environment_lib/Environment/Driver/SPEED_PROFILER  Tag=ASM_SUBCOMPONENT  ASMProperties=struct('Name','SPEED_PROFILER','Version','5.0','Library','ASM_Environment_lib')  ASMInstanceName=speed_profiler  ASMInstanceID=1
  Sw_Observe_v_Scenery_Lim[1Off|2On] : Constant  Value=2
  Terminator : Terminator
  Terminator1 : Terminator
  Terminator2 : Terminator
  UnitConversion1 : ASM_Utils_lib/UnitConversion/UnitConversion  Selection=km/h_to_m/s
  a_z_Max_Deflect[m|s2] : Constant  Value=2.5
  a_z_Max_Rebound[m|s2] : Constant  Value=-3.5
  n_GG_Acceleration[-] : Constant  Value=2
  n_GG_Deceleration[-] : Constant  Value=2
  v_x_Ref_OutsideRoad[m|s] : Constant  Value=2.78
  v_Vehicle_Ref[m|s] : Outport  VectorParamsAs1DForOutWhenUnconnected=off
  v_Vehicle_Ref_Preview[m|s] : Outport  Port=2  VectorParamsAs1DForOutWhenUnconnected=off
  s_Preview_vRef[m] : Outport  Port=3  VectorParamsAs1DForOutWhenUnconnected=off
  tag scope: ASMBUS_Driver_Curvature=scoped, ASMBUS_Driver_SpeedProfiler=scoped
  wires:
  AdaptationForNegativeSpeed/1(Out1) -> SPEED_PROFILER/10
  Bus Selector4/16 -> SPEED_PROFILER/18  "<a_x_Vehicle_Ref_TrafficDriver[m|s2]>"
  Bus Selector4/15 -> SPEED_PROFILER/17  "<Mode_TrafficDriver[1Off|2On]>"
  Bus Selector4/14 -> SPEED_PROFILER/16  "<Reset_States[0|1]>"
  Bus Selector4/13 -> SPEED_PROFILER/15  "<Route_Direction_Init[]>"
  Bus Selector4/12 -> SPEED_PROFILER/14  "<s_Vehicle_Init[m]>"
  Bus Selector4/11 -> SPEED_PROFILER/13  "<v_Vehicle_Preview_Ref_Maneuver[m|s]>"
  Bus Selector4/10 -> SPEED_PROFILER/12, AdaptationForNegativeSpeed/2(v_Vehicle_Ref_Maneuver[km|h])  "<v_Vehicle_Ref_Maneuver[m|s]>"
  Bus Selector4/9 -> SPEED_PROFILER/11  "<Mode_AcceleratorBrake[1Stim|2Driver]>"
  Bus Selector4/8 -> AdaptationForNegativeSpeed/1(Mode_AdaptVelocityToRoad[1Off|2On])  "<Mode_AdaptVelocityToRoad[1Off|2On]>"
  Bus Selector2/1 -> DRIVER_CURVATURE/1  "<Mode_CurvatureCalculation[1Road|2Driver]>"
  Bus Selector2/2 -> DRIVER_CURVATURE/2  "<Pos_x_Preview_DriverCurv[m]>"
  Bus Selector2/3 -> DRIVER_CURVATURE/3  "<Pos_y_Preview_DriverCurv[m]>"
  Bus Selector2/4 -> DRIVER_CURVATURE/4  "<Curv_Veh_Road[1|m]>"
  Bus Selector2/5 -> Reduce_Dimension3/1(In)  "<Curv_Preview_Road[1|m]>"
  Bus Selector4/7 -> SPEED_PROFILER/9  "<Dist_Border_Right[m]>"
  Bus Selector4/6 -> SPEED_PROFILER/8  "<Dist_Border_Left[m]>"
  Bus Selector4/5 -> Reduce_Dimension1/1(In)  "<Pos_z_Preview_Road[m]>"
  Bus Selector4/4 -> Reduce_Dimension/1(In)  "<Pitch_Preview_Road[deg]>"
  Bus Selector4/3 -> Reduce_Dimension2/1(In)  "<Speed_Limit_Preview_Road[km|h]>"
  Bus Selector4/2 -> SPEED_PROFILER/4  "<s_Total_Vehicle_Road[m]>"
  Bus Selector4/1 -> UnitConversion1/1  "<v_x_Vehicle[km|h]>"
  Bus Selector3/1 -> Driver_Parameters/1(a_x_Max[m|s2])  "<a_x_Max[m|s2]>"
  Bus Selector3/2 -> Driver_Parameters/2(a_x_Min[m|s2])  "<a_x_Min[m|s2]>"
  Bus Selector3/3 -> Driver_Parameters/3(a_y_Max[m|s2])  "<a_y_Max[m|s2]>"
  Interface_In/1 -> Bus Selector2/1, Bus Selector3/1, Bus Selector4/1
  Reduce_Dimension4/1(Out) -> SPEED_PROFILER/1
  SPEED_PROFILER/4 -> Terminator1/1
  SPEED_PROFILER/1 -> [ASMBUS_Driver_SpeedProfiler]
  DRIVER_CURVATURE/2 -> Terminator2/1
  t_Preview_vRef[s]/1 -> Driver_Parameters/8(t_Preview_vRef[s])
  Reduce_Dimension1/1(Out) -> SPEED_PROFILER/7
  Reduce_Dimension/1(Out) -> SPEED_PROFILER/6
  SPEED_PROFILER/3 -> v_Vehicle_Ref_Preview[m|s]/1
  SPEED_PROFILER/2 -> v_Vehicle_Ref[m|s]/1
  Extend_Previews/1(Out) -> s_Preview_vRef[m]/1
  SPEED_PROFILER/5 -> Terminator/1
  n_GG_Deceleration[-]/1 -> Driver_Parameters/5(n_GG_Deceleration[-])
  n_GG_Acceleration[-]/1 -> Driver_Parameters/4(n_GG_Acceleration[-])
  v_x_Ref_OutsideRoad[m|s]/1 -> Driver_Parameters/10(v_x_Ref_OutsideRoad[m|s])
  Dist_OutsideRoad_Margin[m]/1 -> Driver_Parameters/9(Dist_OutsideRoad_Margin[m])
  a_z_Max_Rebound[m|s2]/1 -> Driver_Parameters/7(a_z_Max_Rebound[m|s2])
  a_z_Max_Deflect[m|s2]/1 -> Driver_Parameters/6(a_z_Max_Deflect[m|s2])
  Reduce_Dimension2/1(Out) -> SPEED_PROFILER/5
  Driver_Parameters/1(Driver_Parameters) -> SPEED_PROFILER/2
  UnitConversion1/1 -> SPEED_PROFILER/3
  SPEED_PROFILER/6 -> Extend_Previews/1(In)
  DRIVER_CURVATURE/3 -> Reduce_Dimension4/1(In)
  DRIVER_CURVATURE/1 -> [ASMBUS_Driver_Curvature]
  Reduce_Dimension3/1(Out) -> DRIVER_CURVATURE/5
  Sw_Observe_v_Scenery_Lim[1Off|2On]/1 -> Driver_Parameters/11(Sw_Observe_v_Scenery_Lim[1Off|2On])
  Bus Selector4/17 -> SPEED_PROFILER/19  "<Enable_v_Init[0|1]>"
  Bus Selector4/18 -> SPEED_PROFILER/20  "<Lane_ID_Vehicle[]>"

== system ASM_Traffic_A11/Driver/Plant/UserInterface/ASMSignalBus_Plant ==
  In : Inport
  Terminator_1 : Terminator
  tag scope: ASMBUS_Driver_Plant=global
  wires:
  [ASMBUS_Driver_Plant] -> Terminator_1/1
  In/1 -> [ASMBUS_Driver_Plant]  "Plant"
